simulink model "Data_Login_E3"  (Simulink 7.0)
settings: Solver=FixedStepDiscrete  StartTime=0.0  StopTime=10.0  FixedStep=0.001  RelTol=1e-3
libraries: dsPICdrivers x6
settings Model: Creator=Lubin  LastModifiedBy=Admin
settings OptimizationCC: OptimizeModelRefInitCode=on  LifeSpan=1
settings DebuggingCC: SaveWithParameterizedLinksMsg=none  SignalResolutionControl=TryResolveAllWithWarning
settings HardwareCC: ProdBitPerInt=16  ProdEndianess=LittleEndian  ProdWordSize=16  ProdHWDeviceType=16-bit Generic  TargetHWDeviceType=32-bit Generic
settings RTWCC: SystemTargetFile=dspic.tlc  MakeCommand=make_CreateMPLAB  TemplateMakefile=dspic_pic30_gcc.tmf  PostCodeGenCommand=dsPIC_Compile()  Description=Embedded Target for Microchip dsPIC (real-time)  ProcessScript=dspic_make_rtw_hook
settings CodeAppCC: IgnoreCustomStorageClasses=off
settings STFCustomTargetCC: TargetFcnLib=ansi_tfl_tmw.mat  GenFloatMathFcnCalls=ANSI_C  IncludeMdlTerminateFcn=off  CombineOutputUpdateFcns=on  SuppressErrorStatus=on  ERTCustomFileBanners=on  SupportAbsoluteTime=off  SupportNonFinite=off  SupportComplex=off  SupportContinuousTime=off  SupportNonInlinedSFcns=off  ModelStepFunctionPrototypeControlCompliant=on  SystemTargetFile=dspic.tlc
settings ERTTargetCC: TargetFcnLib=ansi_tfl_tmw.mat  GenFloatMathFcnCalls=ANSI_C  CompOptLevelCompliant=off  IncludeMdlTerminateFcn=off  SuppressErrorStatus=on  SupportAbsoluteTime=off  SupportNonFinite=off  SupportComplex=off  ExtModeMexFile=ext_serial_win32_comm  InlinedParameterPlacement=NonHierarchical  ERTSrcFileBannerTemplate=dsPIC_code_template.cgt  ERTHdrFileBannerTemplate=dsPIC_code_template.cgt  ERTDataSrcFileTemplate=dsPIC_code_template.cgt  ERTDataHdrFileTemplate=dsPIC_code_template.cgt  ERTCustomFileTemplate=dsPIC_main.tlc
settings CustomProperty: DataType=string  Value=C:\PROGRA~1\MATLAB\R2007b\bin\win32\gmake

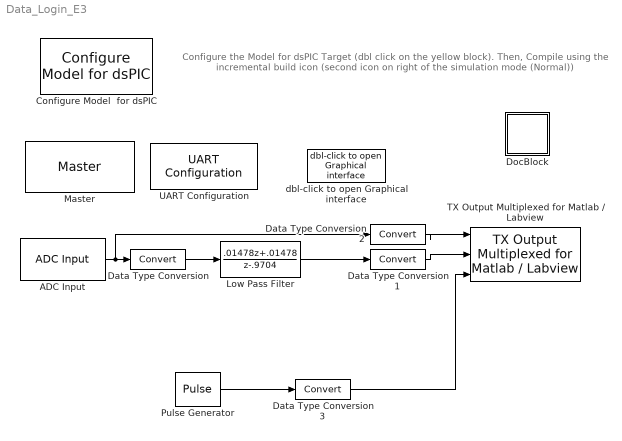
== system Data_Login_E3 ==
  note: Configure the Model for dsPIC Target (dbl click on the yellow block).
      | Then, Compile using the incremental build icon
      | (second icon on right of the simulation mode (Normal))
  ADC Input : dsPICdrivers/Peripheral I//O/ADC Input  Tag=dsPIC_ADC  Priority=5  ADC_TYPE=10 bits  ADC_MODE=Continuous sampling & get last channel value  NbrSampleStep=1  VoltRefpopup="AVdd  -  AVss"  OutFormatBitspopup=0000 00dd dddd dddd : Integer  InterruptPriority=6  ANCHANNELS=[5]  MaxName=ANmax = 1023  Rin=5e6  ADCS=4  SAMC=31  Temperature=25  DMAChannel=0  SampleTime=.001  Status="OK  |  Tsmp=4.844e-006 |  T/Channel=6.719e-006 |  Tall=6.719e-006"  SSRC=auto convert
  Configure Model  for dsPIC : dsPICdrivers/Simulink Configuration/Configure Model  for dsPIC
  Data Type Conversion : DataTypeConversion  OutDataTypeMode=double  OutDataType=sfix(16)  OutScaling=2^0
  Data Type Conversion1 : DataTypeConversion  OutDataTypeMode=uint16  OutDataType=sfix(16)  OutScaling=2^0
  Data Type Conversion2 : DataTypeConversion  OutDataTypeMode=uint16  OutDataType=sfix(16)  OutScaling=2^0
  Data Type Conversion3 : DataTypeConversion  OutDataTypeMode=uint16  OutDataType=sfix(16)  OutScaling=2^0
  DocBlock : Subsystem
      settings: AttributesFormatString=Clock to open web page\nabout this model  OpenFcn=stat = web('http://www.kerhuel.eu/wiki/Animation_Log_and_Plot_datas_from_PIC_with_Matlab#5', '-browser')
      mask Type: WWW Link
      mask Display:
      | plot([.8 0 0 1 1 .8 .8 1],[1 1 0 0 .8 1 .8 .8]);
      | text(.5,.6,'http://','horizontalalignment','center');
      | text(.95,.05,'Link','verticalalignment','bottom','horizontalalignment','right');
  Low Pass Filter : DiscreteTransferFcn  Numerator=[.01478 .01478]  Denominator=[1 -.9704]  SampleTime=.001
  Master : dsPICdrivers/Master  Tag=dsPIC_MASTER  Priority=1  TimeStepType=Timer1  picType=24fJ128GA010  fcy=16000000  Quartz_33f=8e6  PLLActive_33f=on  fcyDesired_33f=0  tmr1="[1  15999  0]"  tmr1Info="Time Step : 0.001  ;   Error : 0%  PR1=15999"  tmr2345="[0  0  0  0]"  tmr2345cfg=[-1 -1 -1 -1]  IOautoConf=on  typePort="[ 0  0  0  0  0  0  0  0  0  0  0  0  0  0  0  0  0  0  0  0  0  8  0  0  0  0  0  0  0  0  0  0  0  0  0  0  0  0  0  0  0  0  0  0  0  0  0  0  0  0  0  0  0  0  0  0  0  0  0  0  0  0  0  0  0  0  0  0  0  0  0  0  0  0  0  0  0  0  0  0  0  0  0  0  4  5  0  0  0  0  0  0  0  0  0  0  0  0  0  0  0  0  0  0  0  0  0  0  0  0  0  0 ]"  TRIS="[ 65535  65535  65535  65535  65535  65535  65535 ]"  ADPCFG=0  MasterBusyPort=None  MasterOverloadPort=None  FOSC=Quartz (XT - HS)  ClockSwitchMonitor=Both disabled  TempProtection_33f=TEMP_ON  FPBOR=<empty>  PWRT=disable  MCLR=<empty>  ICD=ICS_PGD1  JTAGEN=JTAGEN_OFF  PowerSave=off  OverrideFcy=off  NewFcy=1e6  PR2345="[65535  65535  65535  65535]"
  Pulse Generator : DiscretePulseGenerator  Amplitude=500  Period=1000  PulseWidth=500  SampleTime=.001
  TX Output Multiplexed for Matlab / Labview : dsPICdrivers/Serial PORT/TX Output Multiplexed for Matlab // Labview  Tag=dsPIC_TX_Multiplexed  Priority=5  UART=2  CleverSpreadingChk=on  CleverSpreading=1  CHANNEL=[0 1 2]  CHANNELBLOCKED=[]  CHANNELBLOCKED_BITEWISE=0  Status=OK
  UART Configuration : dsPICdrivers/Serial PORT/UART Configuration  Tag=dsPIC_config_UART  Priority=2  UART=2  proposed_BAUD=115200  BAUD=115200  ALT_TX_RX=on  InterruptTxWhen=When Transmit Buffer is empty  TXInterruptPri=1  TxBufferSize=32  TXEN=on  InterruptRxWhen=When Receive Buffer is full (contain 4 characters)  RXInterruptPri=1  RxBufferSize=32  UxBRG=8  Info="UxBRG = 8   ||  Real Baud : 111111   ||  % error : -3.5494  ||  max 11.1111 Bytes / Step"  RealBaud=0  ERROR=-3.5494  BYTES_STEP=11.1111
  dbl-click to open Graphical interface : dsPICdrivers/Serial PORT/dbl-click to open Graphical interface  Nothing=0
  wires:
  Data Type Conversion2/1 -> TX Output Multiplexed for Matlab / Labview/1
  Data Type Conversion1/1 -> TX Output Multiplexed for Matlab / Labview/2
  Low Pass Filter/1 -> Data Type Conversion1/1
  Data Type Conversion/1 -> Low Pass Filter/1
  ADC Input/1 -> Data Type Conversion/1, Data Type Conversion2/1
  Pulse Generator/1 -> Data Type Conversion3/1
  Data Type Conversion3/1 -> TX Output Multiplexed for Matlab / Labview/3

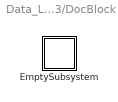
== system Data_Login_E3/DocBlock ==
  EmptySubsystem : Subsystem

== system Data_Login_E3/DocBlock/EmptySubsystem ==
